simulink model "trucksim_specific_control_with_rule_model"  (R2023b)
settings: Solver=FixedStepAuto  StartTime=0.0  StopTime=25  FixedStep=0.001  RelTol=1e-3  EnableMultiTasking=on
values from neighbouring files (symbols this model uses):
  A = 5    [unlinear_vehicle_Parameters.m]
  Bf = 1.725    [unlinear_vehicle_Parameters.m]
  Br = 1.750    (= 1.75)    [unlinear_vehicle_Parameters.m]
  Cd = 0.4    [unlinear_vehicle_Parameters.m]
  Cs_f = 4302    [unlinear_vehicle_Parameters.m]
  Delta_act_sine_amp = delta_act_sine_amp(j)    [Truck_simulate.m]    (also in unlinear_vehicle_Parameters.m)
  Delta_act_sine_fre = delta_act_sine_fre(k)    [Truck_simulate.m]    (also in unlinear_vehicle_Parameters.m)
  f = 0.01    [unlinear_vehicle_Parameters.m]
  g = 9.8    [Truck_simulate.m]    (also in unlinear_vehicle_Parameters.m)
  He = 0.45    [unlinear_vehicle_Parameters.m]
  hg = 0.781    [unlinear_vehicle_Parameters.m]
  Hp = 0.2    [unlinear_vehicle_Parameters.m]
  I_tire = 0.7    [unlinear_vehicle_Parameters.m]
  Ix = 423.3    [unlinear_vehicle_Parameters.m]
  Iy = 1762.5    [unlinear_vehicle_Parameters.m]
  Iz = 1762.5    [unlinear_vehicle_Parameters.m]
  ks_f = 189000    [unlinear_vehicle_Parameters.m]
  kw = 220000    [unlinear_vehicle_Parameters.m]
  L = 3.140    (= 3.14)    [unlinear_vehicle_Parameters.m]
  Lf = 1.330    (= 1.33)    [unlinear_vehicle_Parameters.m]
  Lr = 3.140 - 1.330    (= 1.81)    [unlinear_vehicle_Parameters.m]
  m = m_sprung + m_load + m_unsprung    (= 10505)    [Truck_simulate.m]    (also in unlinear_vehicle_Parameters.m = 1407.3)
  mb = 1128.5 + 000    (= 1128.5)    [unlinear_vehicle_Parameters.m]
  mw = 139.4 / 2    (= 69.7)    [unlinear_vehicle_Parameters.m]
  p = 1.206    [unlinear_vehicle_Parameters.m]
  r = 0.510    (= 0.51)    [Truck_simulate.m]    (also in unlinear_vehicle_Parameters.m = 0.287)
  T_motor_constant = t_motor_const(i)    [Truck_simulate.m]    (also in unlinear_vehicle_Parameters.m)
  vx0 = 5    [Truck_simulate.m]    (also in unlinear_vehicle_Parameters.m)
  vy0 = 0    [Truck_simulate.m]    (also in unlinear_vehicle_Parameters.m)
  w0 = vx0 / r    (= 9.80392156863)    [Truck_simulate.m]    (also in unlinear_vehicle_Parameters.m = 17.4216027875)
  wz0 = 0    [Truck_simulate.m]    (also in unlinear_vehicle_Parameters.m)
libraries: Solver_SF x1
(part 2 of 4)

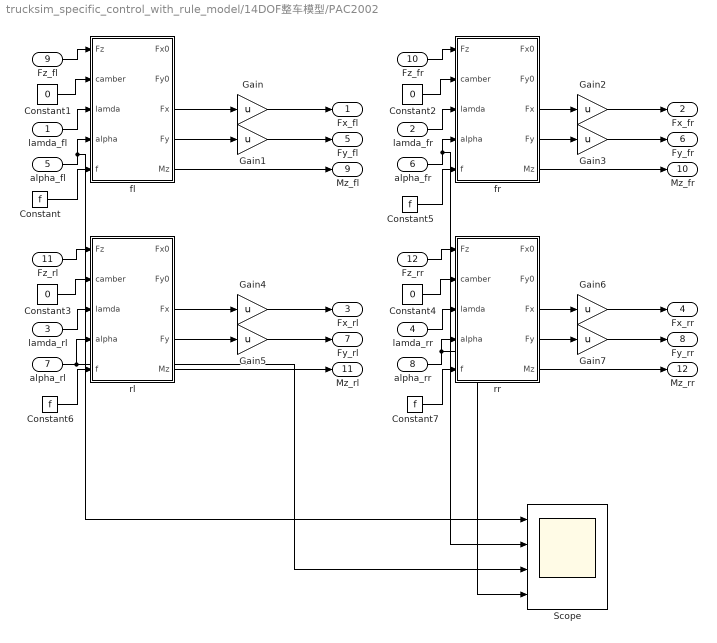
== system trucksim_specific_control_with_rule_model/14DOF整车模型/PAC2002 ==
  lamda_fl : Inport
  lamda_fr : Inport  Port=2
  lamda_rl : Inport  Port=3
  lamda_rr : Inport  Port=4
  alpha_fl : Inport  Port=5
  alpha_fr : Inport  Port=6
  alpha_rl : Inport  Port=7
  alpha_rr : Inport  Port=8
  Fz_fl : Inport  Port=9
  Fz_fr : Inport  Port=10
  Fz_rl : Inport  Port=11
  Fz_rr : Inport  Port=12
  Constant{,5..7} (4 alike) : Constant  Value=f
  Constant{1..4} (4 alike) : Constant  Value=0
  Gain{,1..7} (8 alike) : Gain  Gain=u
  Scope : Scope  NumInputPorts=4
  fl : MATLAB Function  TreatAsAtomicUnit=on
  fr : MATLAB Function  TreatAsAtomicUnit=on
  rl : MATLAB Function  TreatAsAtomicUnit=on
  rr : MATLAB Function  TreatAsAtomicUnit=on
  Fx_fl : Outport
  Fx_fr : Outport  Port=2
  Fx_rl : Outport  Port=3
  Fx_rr : Outport  Port=4
  Fy_fl : Outport  Port=5
  Fy_fr : Outport  Port=6
  Fy_rl : Outport  Port=7
  Fy_rr : Outport  Port=8
  Mz_fl : Outport  Port=9
  Mz_fr : Outport  Port=10
  Mz_rl : Outport  Port=11
  Mz_rr : Outport  Port=12
  wires:
  Constant4/1 -> rr/2(camber)
  Constant3/1 -> rl/2(camber)
  Constant2/1 -> fr/2(camber)
  rr/5(Mz) -> Mz_rr/1
  rl/5(Mz) -> Mz_rl/1
  Fz_rr/1 -> rr/1(Fz)
  alpha_rr/1 -> Scope/4, rr/4(alpha)
  lamda_rr/1 -> rr/3(lamda)
  Fz_rl/1 -> rl/1(Fz)
  alpha_rl/1 -> Scope/3, rl/4(alpha)
  lamda_rl/1 -> rl/3(lamda)
  fr/5(Mz) -> Mz_fr/1
  Fz_fr/1 -> fr/1(Fz)
  alpha_fr/1 -> Scope/2, fr/4(alpha)
  lamda_fr/1 -> fr/3(lamda)
  fl/5(Mz) -> Mz_fl/1
  Constant1/1 -> fl/2(camber)
  Fz_fl/1 -> fl/1(Fz)
  alpha_fl/1 -> Scope/1, fl/4(alpha)
  lamda_fl/1 -> fl/3(lamda)
  fl/3(Fx) -> Gain/1
  fl/4(Fy) -> Gain1/1
  fr/4(Fy) -> Gain3/1
  rr/3(Fx) -> Gain6/1
  rr/4(Fy) -> Gain7/1
  rl/3(Fx) -> Gain4/1
  rl/4(Fy) -> Gain5/1
  fr/3(Fx) -> Gain2/1
  Gain/1 -> Fx_fl/1
  Gain1/1 -> Fy_fl/1
  Gain2/1 -> Fx_fr/1
  Gain3/1 -> Fy_fr/1
  Gain4/1 -> Fx_rl/1
  Gain5/1 -> Fy_rl/1
  Gain6/1 -> Fx_rr/1
  Gain7/1 -> Fy_rr/1
  Constant/1 -> fl/5(f)
  Constant5/1 -> fr/5(f)
  Constant6/1 -> rl/5(f)
  Constant7/1 -> rr/5(f)

== system trucksim_specific_control_with_rule_model/14DOF整车模型/Wheel ==
  T_fl : Inport
  T_fr : Inport  Port=2
  T_rl : Inport  Port=3
  T_rr : Inport  Port=4
  Fx_fl : Inport  Port=5
  Fx_fr : Inport  Port=6
  Fx_rl : Inport  Port=7
  Fx_rr : Inport  Port=8
  Fz_fl : Inport  Port=9
  Fz_fr : Inport  Port=10
  Fz_rl : Inport  Port=11
  Fz_rr : Inport  Port=12
  fl : Subsystem
  fr : Subsystem
  rl : Subsystem
  rr : Subsystem
  w_fl : Outport
  w_fr : Outport  Port=2
  w_rl : Outport  Port=3
  w_rr : Outport  Port=4
  wires:
  rr/1(w_rr) -> w_rr/1
  Fz_rr/1 -> rr/3(Fz_rr)
  Fx_rr/1 -> rr/2(Fx_rr)
  T_rr/1 -> rr/1(T_rr)
  rl/1(w_rl) -> w_rl/1
  Fz_rl/1 -> rl/3(Fz_rl)
  Fx_rl/1 -> rl/2(Fx_rl)
  T_rl/1 -> rl/1(T_rl)
  Fz_fr/1 -> fr/3(Fz_fr)
  Fx_fr/1 -> fr/2(Fx_fr)
  T_fr/1 -> fr/1(T_fr)
  fr/1(w_fr) -> w_fr/1
  fl/1(w_fl) -> w_fl/1
  Fz_fl/1 -> fl/3(Fz_fl)
  Fx_fl/1 -> fl/2(Fx_fl)
  T_fl/1 -> fl/1(T_fl)

== system trucksim_specific_control_with_rule_model/14DOF整车模型/alpha_lamda ==
  vx : Inport
  vy : Inport  Port=2
  wz : Inport  Port=3
  delta_fl : Inport  Port=4
  delta_fr : Inport  Port=5
  delta_rl : Inport  Port=6
  delta_rr : Inport  Port=7
  w_fl : Inport  Port=8
  w_fr : Inport  Port=9
  w_rl : Inport  Port=10
  w_rr : Inport  Port=11
  alpha : Subsystem
  lamda : Subsystem
  lamda_fl : Outport
  lamda_fr : Outport  Port=2
  lamda_rl : Outport  Port=3
  lamda_rr : Outport  Port=4
  alpha_fl : Outport  Port=5
  alpha_fr : Outport  Port=6
  alpha_rl : Outport  Port=7
  alpha_rr : Outport  Port=8
  wires:
  alpha/1(alpha_fl) -> alpha_fl/1
  alpha/2(alpha_fr) -> alpha_fr/1
  alpha/3(alpha_rl) -> alpha_rl/1
  alpha/4(alpha_rr) -> alpha_rr/1
  vx/1 -> lamda/1(vx), alpha/1(vx)
  vy/1 -> lamda/2(vy), alpha/2(vy)
  wz/1 -> lamda/3(wz), alpha/3(wz)
  delta_fl/1 -> lamda/4(delta_fl), alpha/4(delta_fl)
  delta_fr/1 -> lamda/5(delta_fr), alpha/5(delta_fr)
  w_fl/1 -> lamda/6(w_fl)
  w_fr/1 -> lamda/7(w_fr)
  w_rl/1 -> lamda/8(w_rl)
  w_rr/1 -> lamda/9(w_rr)
  lamda/1(lamda_fl) -> lamda_fl/1
  lamda/2(lamda_fr) -> lamda_fr/1
  lamda/4(lamda_rr) -> lamda_rr/1
  lamda/3(lamda_rl) -> lamda_rl/1
  delta_rl/1 -> lamda/10(delta_rl), alpha/6(delta_rl)
  delta_rr/1 -> lamda/11(delta_rr), alpha/7(delta_rr)

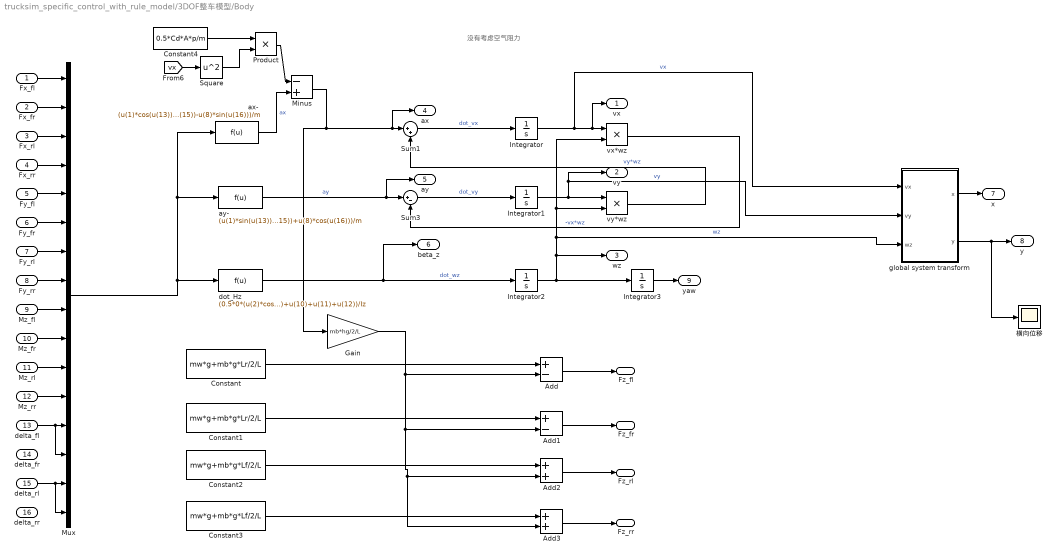
== system trucksim_specific_control_with_rule_model/3DOF整车模型/Body ==
  note: 没有考虑空气阻力
  Fx_fl : Inport
  Fx_fr : Inport  Port=2
  Fx_rl : Inport  Port=3
  Fx_rr : Inport  Port=4
  Fy_fl : Inport  Port=5
  Fy_fr : Inport  Port=6
  Fy_rl : Inport  Port=7
  Fy_rr : Inport  Port=8
  Mz_fl : Inport  Port=9
  Mz_fr : Inport  Port=10
  Mz_rl : Inport  Port=11
  Mz_rr : Inport  Port=12
  delta_fl : Inport  Port=13
  delta_fr : Inport  Port=14
  delta_rl : Inport  Port=15
  delta_rr : Inport  Port=16
  Add : Sum  Inputs=+-
  Add1 : Sum  Inputs=+-
  Add2 : Sum
  Add3 : Sum
  Constant : Constant  Value=mw*g+mb*g*Lr/2/L
  Constant1 : Constant  Value=mw*g+mb*g*Lr/2/L
  Constant2 : Constant  Value=mw*g+mb*g*Lf/2/L
  Constant3 : Constant  Value=mw*g+mb*g*Lf/2/L
  Constant4 : Constant  Value=0.5*Cd*A*p/m
  Gain : Gain  Gain=mb*hg/2/L
  Integrator : Integrator  InitialCondition=vx0  LimitOutput=on  LowerSaturationLimit=0
  Integrator1 : Integrator  InitialCondition=vy0
  Integrator2 : Integrator  InitialCondition=wz0
  Integrator3 : Integrator
  Minus : Sum  Inputs=-+
  Mux : Mux  Inputs=16
  Product : Product
  Square : Math  Operator=square
  Sum1 : Sum  Inputs=|++
  Sum3 : Sum  Inputs=|+-
  ax- : Fcn  Expr=(u(1)*cos(u(13))+u(2)*cos(u(14))-u(5)*sin(u(13))-u(6)*sin(u(14))+u(3)*cos(u(15))+u(4)*cos(u(16))-u(7)*sin(u(15))-u(8)*sin(u(16)))/m
  ay- : Fcn  Expr=(u(1)*sin(u(13))+u(2)*sin(u(14))+u(5)*cos(u(13))+u(6)*cos(u(14))+u(3)*sin(u(15))+u(4)*sin(u(16))+u(7)*cos(u(15))+u(8)*cos(u(16)))/m
  dot_Hz : Fcn  Expr=(0.5*0*(u(2)*cos(u(14))-u(1)*cos(u(13))-u(6)*sin(u(14))+u(5)*sin(u(13)))+0.5*0*(u(4)*cos(u(16))-u(3)*cos(u(15))-u(8)*sin(u(16))+u(7)*sin(u(15)))+Lf*(u(1)*sin(u(13))+u(5)*cos(u(13))+u(2)*sin(u(14))+u(6)*cos(u(14)))-Lr*(u(3)*sin(u(15))+u(7)*cos(u(15))+u(4)*sin(u(16))+u(8)*cos(u(16)))+u(9)+u(10)+u(11)+u(12))/Iz
  global system transform : Subsystem
  vx*wz : Product
  vy*wz : Product
  横向位移 : Scope
  vx : Outport
  vy : Outport  Port=2
  wz : Outport  Port=3
  ax : Outport  Port=4
  ay : Outport  Port=5
  beta_z : Outport  Port=6
  x : Outport  Port=7
  y : Outport  Port=8
  yaw : Outport  Port=9
  Fz_fl : Outport  Port=10
  Fz_fr : Outport  Port=11
  Fz_rl : Outport  Port=12
  Fz_rr : Outport  Port=13
  wires:
  global system transform/2(y) -> y/1, 横向位移/1
  global system transform/1(x) -> x/1
  Mux/1 -> dot_Hz/1, ay-/1, ax-/1
  delta_fl/1 -> Mux/14, Mux/13
  Mz_rr/1 -> Mux/12
  Mz_rl/1 -> Mux/11
  Mz_fr/1 -> Mux/10
  Mz_fl/1 -> Mux/9
  Fy_rr/1 -> Mux/8
  Fy_rl/1 -> Mux/7
  Fy_fr/1 -> Mux/6
  Fy_fl/1 -> Mux/5
  Fx_rr/1 -> Mux/4
  Fx_rl/1 -> Mux/3
  Fx_fr/1 -> Mux/2
  Fx_fl/1 -> Mux/1
  Sum1/1 -> Integrator/1  "dot_vx"
  Integrator/1 -> vx/1, vx*wz/1, global system transform/1(vx)  "vx"
  Integrator1/1 -> global system transform/2(vy), vy/1, vy*wz/1  "vy"
  Sum3/1 -> Integrator1/1  "dot_vy"
  dot_Hz/1 -> beta_z/1, Integrator2/1  "dot_wz"
  Integrator2/1 -> Integrator3/1, global system transform/3(wz), vy*wz/2, vx*wz/2, wz/1  "wz"
  ay-/1 -> ay/1, Sum3/1  "ay"
  vy*wz/1 -> Sum1/2  "vy*wz"
  vx*wz/1 -> Sum3/2  "-vx*wz"
  Constant/1 -> Add/1
  Gain/1 -> Add3/2, Add2/2, Add1/2, Add/2
  Add/1 -> Fz_fl/1
  Constant1/1 -> Add1/1
  Add1/1 -> Fz_fr/1
  Constant2/1 -> Add2/1
  Add2/1 -> Fz_rl/1
  Constant3/1 -> Add3/1
  Add3/1 -> Fz_rr/1
  Constant4/1 -> Product/1
  Square/1 -> Product/2
  [vx] -> Square/1
  Product/1 -> Minus/1
  ax-/1 -> Minus/2  "ax"
  Minus/1 -> Gain/1, ax/1, Sum1/1
  delta_rl/1 -> Mux/16, Mux/15
  Integrator3/1 -> yaw/1

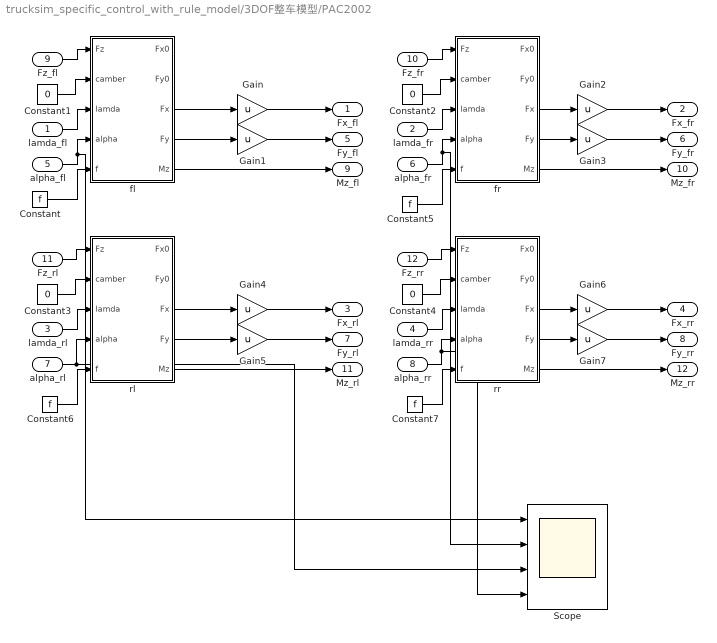
== system trucksim_specific_control_with_rule_model/3DOF整车模型/PAC2002 ==
  lamda_fl : Inport
  lamda_fr : Inport  Port=2
  lamda_rl : Inport  Port=3
  lamda_rr : Inport  Port=4
  alpha_fl : Inport  Port=5
  alpha_fr : Inport  Port=6
  alpha_rl : Inport  Port=7
  alpha_rr : Inport  Port=8
  Fz_fl : Inport  Port=9
  Fz_fr : Inport  Port=10
  Fz_rl : Inport  Port=11
  Fz_rr : Inport  Port=12
  Constant{,5..7} (4 alike) : Constant  Value=f
  Constant{1..4} (4 alike) : Constant  Value=0
  Gain{,1..7} (8 alike) : Gain  Gain=u
  Scope : Scope  NumInputPorts=4
  fl : MATLAB Function  TreatAsAtomicUnit=on
  fr : MATLAB Function  TreatAsAtomicUnit=on
  rl : MATLAB Function  TreatAsAtomicUnit=on
  rr : MATLAB Function  TreatAsAtomicUnit=on
  Fx_fl : Outport
  Fx_fr : Outport  Port=2
  Fx_rl : Outport  Port=3
  Fx_rr : Outport  Port=4
  Fy_fl : Outport  Port=5
  Fy_fr : Outport  Port=6
  Fy_rl : Outport  Port=7
  Fy_rr : Outport  Port=8
  Mz_fl : Outport  Port=9
  Mz_fr : Outport  Port=10
  Mz_rl : Outport  Port=11
  Mz_rr : Outport  Port=12
  wires:
  Constant4/1 -> rr/2(camber)
  Constant3/1 -> rl/2(camber)
  Constant2/1 -> fr/2(camber)
  rr/5(Mz) -> Mz_rr/1
  rl/5(Mz) -> Mz_rl/1
  Fz_rr/1 -> rr/1(Fz)
  alpha_rr/1 -> Scope/4, rr/4(alpha)
  lamda_rr/1 -> rr/3(lamda)
  Fz_rl/1 -> rl/1(Fz)
  alpha_rl/1 -> Scope/3, rl/4(alpha)
  lamda_rl/1 -> rl/3(lamda)
  fr/5(Mz) -> Mz_fr/1
  Fz_fr/1 -> fr/1(Fz)
  alpha_fr/1 -> Scope/2, fr/4(alpha)
  lamda_fr/1 -> fr/3(lamda)
  fl/5(Mz) -> Mz_fl/1
  Constant1/1 -> fl/2(camber)
  Fz_fl/1 -> fl/1(Fz)
  alpha_fl/1 -> Scope/1, fl/4(alpha)
  lamda_fl/1 -> fl/3(lamda)
  fl/3(Fx) -> Gain/1
  fl/4(Fy) -> Gain1/1
  fr/4(Fy) -> Gain3/1
  rr/3(Fx) -> Gain6/1
  rr/4(Fy) -> Gain7/1
  rl/3(Fx) -> Gain4/1
  rl/4(Fy) -> Gain5/1
  fr/3(Fx) -> Gain2/1
  Gain/1 -> Fx_fl/1
  Gain1/1 -> Fy_fl/1
  Gain2/1 -> Fx_fr/1
  Gain3/1 -> Fy_fr/1
  Gain4/1 -> Fx_rl/1
  Gain5/1 -> Fy_rl/1
  Gain6/1 -> Fx_rr/1
  Gain7/1 -> Fy_rr/1
  Constant/1 -> fl/5(f)
  Constant5/1 -> fr/5(f)
  Constant6/1 -> rl/5(f)
  Constant7/1 -> rr/5(f)

== system trucksim_specific_control_with_rule_model/3DOF整车模型/Wheel ==
  T_fl : Inport
  T_fr : Inport  Port=2
  T_rl : Inport  Port=3
  T_rr : Inport  Port=4
  Fx_fl : Inport  Port=5
  Fx_fr : Inport  Port=6
  Fx_rl : Inport  Port=7
  Fx_rr : Inport  Port=8
  Fz_fl : Inport  Port=9
  Fz_fr : Inport  Port=10
  Fz_rl : Inport  Port=11
  Fz_rr : Inport  Port=12
  fl : Subsystem
  fr : Subsystem
  rl : Subsystem
  rr : Subsystem
  w_fl : Outport
  w_fr : Outport  Port=2
  w_rl : Outport  Port=3
  w_rr : Outport  Port=4
  wires:
  T_fl/1 -> fl/1(T_fl)
  Fx_fl/1 -> fl/2(Fx_fl)
  Fz_fl/1 -> fl/3(Fz_fl)
  fl/1(w_fl) -> w_fl/1
  fr/1(w_fr) -> w_fr/1
  T_fr/1 -> fr/1(T_fr)
  Fx_fr/1 -> fr/2(Fx_fr)
  Fz_fr/1 -> fr/3(Fz_fr)
  T_rl/1 -> rl/1(T_rl)
  Fx_rl/1 -> rl/2(Fx_rl)
  Fz_rl/1 -> rl/3(Fz_rl)
  rl/1(w_rl) -> w_rl/1
  T_rr/1 -> rr/1(T_rr)
  Fx_rr/1 -> rr/2(Fx_rr)
  Fz_rr/1 -> rr/3(Fz_rr)
  rr/1(w_rr) -> w_rr/1

== system trucksim_specific_control_with_rule_model/3DOF整车模型/alpha_lamda1 ==
  vx : Inport
  vy : Inport  Port=2
  wz : Inport  Port=3
  delta_fl : Inport  Port=4
  delta_fr : Inport  Port=5
  delta_rl : Inport  Port=6
  delta_rr : Inport  Port=7
  w_fl : Inport  Port=8
  w_fr : Inport  Port=9
  w_rl : Inport  Port=10
  w_rr : Inport  Port=11
  alpha : Subsystem
  lamda : Subsystem
  lamda_fl : Outport
  lamda_fr : Outport  Port=2
  lamda_rl : Outport  Port=3
  lamda_rr : Outport  Port=4
  alpha_fl : Outport  Port=5
  alpha_fr : Outport  Port=6
  alpha_rl : Outport  Port=7
  alpha_rr : Outport  Port=8
  wires:
  alpha/1(alpha_fl) -> alpha_fl/1
  alpha/2(alpha_fr) -> alpha_fr/1
  alpha/3(alpha_rl) -> alpha_rl/1
  alpha/4(alpha_rr) -> alpha_rr/1
  vx/1 -> lamda/1(vx), alpha/1(vx)
  vy/1 -> lamda/2(vy), alpha/2(vy)
  wz/1 -> lamda/3(wz), alpha/3(wz)
  delta_fl/1 -> lamda/4(delta_fl), alpha/4(delta_fl)
  delta_fr/1 -> lamda/5(delta_fr), alpha/5(delta_fr)
  w_fl/1 -> lamda/6(w_fl)
  w_fr/1 -> lamda/7(w_fr)
  w_rl/1 -> lamda/8(w_rl)
  w_rr/1 -> lamda/9(w_rr)
  lamda/1(lamda_fl) -> lamda_fl/1
  lamda/2(lamda_fr) -> lamda_fr/1
  lamda/4(lamda_rr) -> lamda_rr/1
  lamda/3(lamda_rl) -> lamda_rl/1
  delta_rl/1 -> lamda/10(delta_rl), alpha/6(delta_rl)
  delta_rr/1 -> lamda/11(delta_rr), alpha/7(delta_rr)

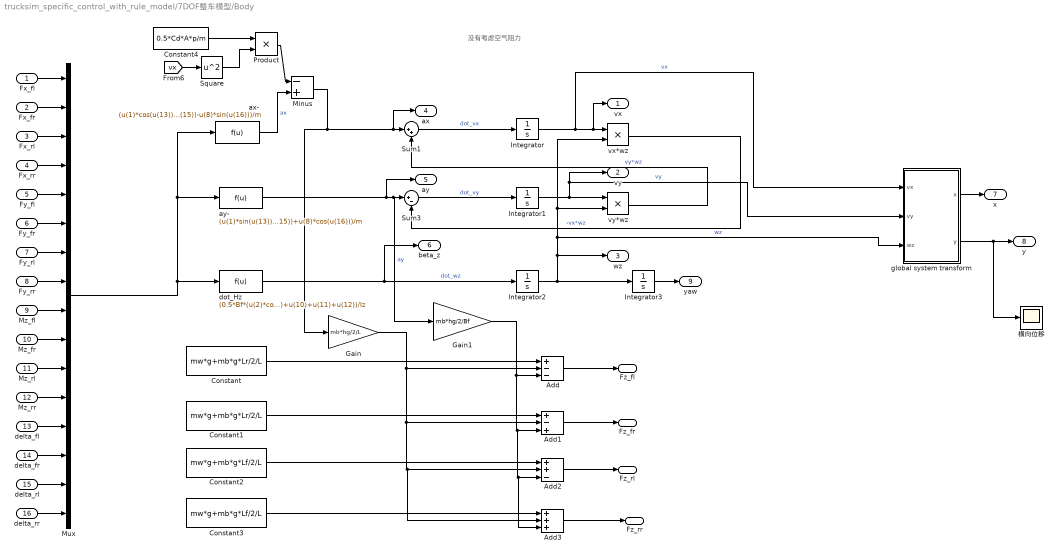
== system trucksim_specific_control_with_rule_model/7DOF整车模型/Body ==
  note: 没有考虑空气阻力
  Fx_fl : Inport
  Fx_fr : Inport  Port=2
  Fx_rl : Inport  Port=3
  Fx_rr : Inport  Port=4
  Fy_fl : Inport  Port=5
  Fy_fr : Inport  Port=6
  Fy_rl : Inport  Port=7
  Fy_rr : Inport  Port=8
  Mz_fl : Inport  Port=9
  Mz_fr : Inport  Port=10
  Mz_rl : Inport  Port=11
  Mz_rr : Inport  Port=12
  delta_fl : Inport  Port=13
  delta_fr : Inport  Port=14
  delta_rl : Inport  Port=15
  delta_rr : Inport  Port=16
  Add : Sum  Inputs=+--
  Add1 : Sum  Inputs=+-+
  Add2 : Sum  Inputs=++-
  Add3 : Sum  Inputs=+++
  Constant : Constant  Value=mw*g+mb*g*Lr/2/L
  Constant1 : Constant  Value=mw*g+mb*g*Lr/2/L
  Constant2 : Constant  Value=mw*g+mb*g*Lf/2/L
  Constant3 : Constant  Value=mw*g+mb*g*Lf/2/L
  Constant4 : Constant  Value=0.5*Cd*A*p/m
  Gain : Gain  Gain=mb*hg/2/L
  Gain1 : Gain  Gain=mb*hg/2/Bf
  Integrator : Integrator  InitialCondition=vx0  LimitOutput=on  LowerSaturationLimit=0
  Integrator1 : Integrator  InitialCondition=vy0
  Integrator2 : Integrator  InitialCondition=wz0
  Integrator3 : Integrator
  Minus : Sum  Inputs=-+
  Mux : Mux  Inputs=16
  Product : Product
  Square : Math  Operator=square
  Sum1 : Sum  Inputs=|++
  Sum3 : Sum  Inputs=|+-
  ax- : Fcn  Expr=(u(1)*cos(u(13))+u(2)*cos(u(14))-u(5)*sin(u(13))-u(6)*sin(u(14))+u(3)*cos(u(15))+u(4)*cos(u(16))-u(7)*sin(u(15))-u(8)*sin(u(16)))/m
  ay- : Fcn  Expr=(u(1)*sin(u(13))+u(2)*sin(u(14))+u(5)*cos(u(13))+u(6)*cos(u(14))+u(3)*sin(u(15))+u(4)*sin(u(16))+u(7)*cos(u(15))+u(8)*cos(u(16)))/m
  dot_Hz : Fcn  Expr=(0.5*Bf*(u(2)*cos(u(14))-u(1)*cos(u(13))-u(6)*sin(u(14))+u(5)*sin(u(13)))+0.5*Br*(u(4)*cos(u(16))-u(3)*cos(u(15))-u(8)*sin(u(16))+u(7)*sin(u(15)))+Lf*(u(1)*sin(u(13))+u(5)*cos(u(13))+u(2)*sin(u(14))+u(6)*cos(u(14)))-Lr*(u(3)*sin(u(15))+u(7)*cos(u(15))+u(4)*sin(u(16))+u(8)*cos(u(16)))+u(9)+u(10)+u(11)+u(12))/Iz
  global system transform : Subsystem
  vx*wz : Product
  vy*wz : Product
  横向位移 : Scope
  vx : Outport
  vy : Outport  Port=2
  wz : Outport  Port=3
  ax : Outport  Port=4
  ay : Outport  Port=5
  beta_z : Outport  Port=6
  x : Outport  Port=7
  y : Outport  Port=8
  yaw : Outport  Port=9
  Fz_fl : Outport  Port=10
  Fz_fr : Outport  Port=11
  Fz_rl : Outport  Port=12
  Fz_rr : Outport  Port=13
  wires:
  global system transform/2(y) -> y/1, 横向位移/1
  global system transform/1(x) -> x/1
  Mux/1 -> dot_Hz/1, ay-/1, ax-/1
  delta_fr/1 -> Mux/14
  delta_fl/1 -> Mux/13
  Mz_rr/1 -> Mux/12
  Mz_rl/1 -> Mux/11
  Mz_fr/1 -> Mux/10
  Mz_fl/1 -> Mux/9
  Fy_rr/1 -> Mux/8
  Fy_rl/1 -> Mux/7
  Fy_fr/1 -> Mux/6
  Fy_fl/1 -> Mux/5
  Fx_rr/1 -> Mux/4
  Fx_rl/1 -> Mux/3
  Fx_fr/1 -> Mux/2
  Fx_fl/1 -> Mux/1
  Sum1/1 -> Integrator/1  "dot_vx"
  Integrator/1 -> vx/1, vx*wz/1, global system transform/1(vx)  "vx"
  Integrator1/1 -> global system transform/2(vy), vy/1, vy*wz/1  "vy"
  Sum3/1 -> Integrator1/1  "dot_vy"
  dot_Hz/1 -> beta_z/1, Integrator2/1  "dot_wz"
  Integrator2/1 -> Integrator3/1, global system transform/3(wz), vy*wz/2, vx*wz/2, wz/1  "wz"
  ay-/1 -> Gain1/1, Sum3/1, ay/1  "ay"
  vy*wz/1 -> Sum1/2  "vy*wz"
  vx*wz/1 -> Sum3/2  "-vx*wz"
  Constant/1 -> Add/1
  Gain/1 -> Add3/2, Add2/2, Add1/2, Add/2
  Gain1/1 -> Add3/3, Add2/3, Add1/3, Add/3
  Add/1 -> Fz_fl/1
  Constant1/1 -> Add1/1
  Add1/1 -> Fz_fr/1
  Constant2/1 -> Add2/1
  Add2/1 -> Fz_rl/1
  Constant3/1 -> Add3/1
  Add3/1 -> Fz_rr/1
  Constant4/1 -> Product/1
  Square/1 -> Product/2
  [vx] -> Square/1
  Product/1 -> Minus/1
  ax-/1 -> Minus/2  "ax"
  Minus/1 -> Gain/1, ax/1, Sum1/1
  delta_rr/1 -> Mux/16
  delta_rl/1 -> Mux/15
  Integrator3/1 -> yaw/1

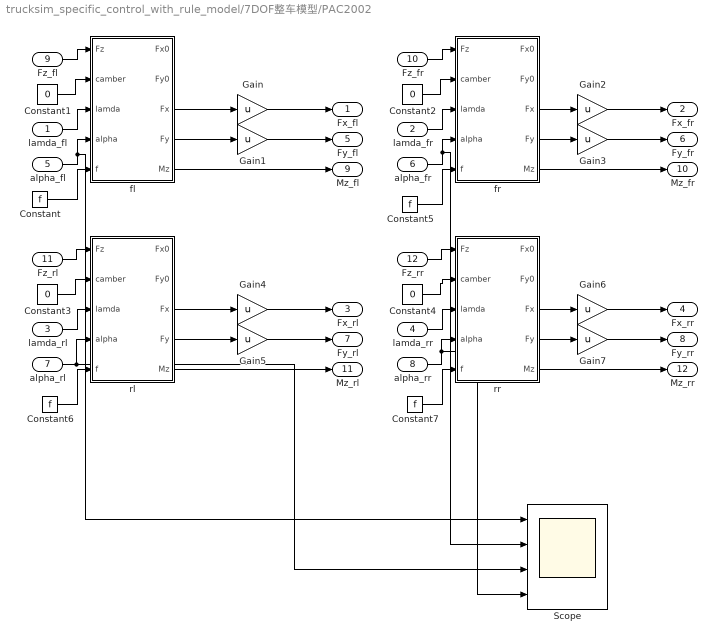
== system trucksim_specific_control_with_rule_model/7DOF整车模型/PAC2002 ==
  lamda_fl : Inport
  lamda_fr : Inport  Port=2
  lamda_rl : Inport  Port=3
  lamda_rr : Inport  Port=4
  alpha_fl : Inport  Port=5
  alpha_fr : Inport  Port=6
  alpha_rl : Inport  Port=7
  alpha_rr : Inport  Port=8
  Fz_fl : Inport  Port=9
  Fz_fr : Inport  Port=10
  Fz_rl : Inport  Port=11
  Fz_rr : Inport  Port=12
  Constant{,5..7} (4 alike) : Constant  Value=f
  Constant{1..4} (4 alike) : Constant  Value=0
  Gain{,1..7} (8 alike) : Gain  Gain=u
  Scope : Scope  NumInputPorts=4
  fl : MATLAB Function  TreatAsAtomicUnit=on
  fr : MATLAB Function  TreatAsAtomicUnit=on
  rl : MATLAB Function  TreatAsAtomicUnit=on
  rr : MATLAB Function  TreatAsAtomicUnit=on
  Fx_fl : Outport
  Fx_fr : Outport  Port=2
  Fx_rl : Outport  Port=3
  Fx_rr : Outport  Port=4
  Fy_fl : Outport  Port=5
  Fy_fr : Outport  Port=6
  Fy_rl : Outport  Port=7
  Fy_rr : Outport  Port=8
  Mz_fl : Outport  Port=9
  Mz_fr : Outport  Port=10
  Mz_rl : Outport  Port=11
  Mz_rr : Outport  Port=12
  wires:
  Constant4/1 -> rr/2(camber)
  Constant3/1 -> rl/2(camber)
  Constant2/1 -> fr/2(camber)
  rr/5(Mz) -> Mz_rr/1
  rl/5(Mz) -> Mz_rl/1
  Fz_rr/1 -> rr/1(Fz)
  alpha_rr/1 -> rr/4(alpha), Scope/4
  lamda_rr/1 -> rr/3(lamda)
  Fz_rl/1 -> rl/1(Fz)
  alpha_rl/1 -> Scope/3, rl/4(alpha)
  lamda_rl/1 -> rl/3(lamda)
  fr/5(Mz) -> Mz_fr/1
  Fz_fr/1 -> fr/1(Fz)
  alpha_fr/1 -> Scope/2, fr/4(alpha)
  lamda_fr/1 -> fr/3(lamda)
  fl/5(Mz) -> Mz_fl/1
  Constant1/1 -> fl/2(camber)
  Fz_fl/1 -> fl/1(Fz)
  alpha_fl/1 -> Scope/1, fl/4(alpha)
  lamda_fl/1 -> fl/3(lamda)
  fl/3(Fx) -> Gain/1
  fl/4(Fy) -> Gain1/1
  fr/4(Fy) -> Gain3/1
  rr/3(Fx) -> Gain6/1
  rr/4(Fy) -> Gain7/1
  rl/3(Fx) -> Gain4/1
  rl/4(Fy) -> Gain5/1
  fr/3(Fx) -> Gain2/1
  Gain/1 -> Fx_fl/1
  Gain1/1 -> Fy_fl/1
  Gain2/1 -> Fx_fr/1
  Gain3/1 -> Fy_fr/1
  Gain4/1 -> Fx_rl/1
  Gain5/1 -> Fy_rl/1
  Gain6/1 -> Fx_rr/1
  Gain7/1 -> Fy_rr/1
  Constant/1 -> fl/5(f)
  Constant5/1 -> fr/5(f)
  Constant6/1 -> rl/5(f)
  Constant7/1 -> rr/5(f)

== system trucksim_specific_control_with_rule_model/7DOF整车模型/Wheel ==
  T_fl : Inport
  T_fr : Inport  Port=2
  T_rl : Inport  Port=3
  T_rr : Inport  Port=4
  Fx_fl : Inport  Port=5
  Fx_fr : Inport  Port=6
  Fx_rl : Inport  Port=7
  Fx_rr : Inport  Port=8
  Fz_fl : Inport  Port=9
  Fz_fr : Inport  Port=10
  Fz_rl : Inport  Port=11
  Fz_rr : Inport  Port=12
  fl : Subsystem
  fr : Subsystem
  rl : Subsystem
  rr : Subsystem
  w_fl : Outport
  w_fr : Outport  Port=2
  w_rl : Outport  Port=3
  w_rr : Outport  Port=4
  wires:
  T_fl/1 -> fl/1(T_fl)
  Fx_fl/1 -> fl/2(Fx_fl)
  Fz_fl/1 -> fl/3(Fz_fl)
  fl/1(w_fl) -> w_fl/1
  fr/1(w_fr) -> w_fr/1
  T_fr/1 -> fr/1(T_fr)
  Fx_fr/1 -> fr/2(Fx_fr)
  Fz_fr/1 -> fr/3(Fz_fr)
  T_rl/1 -> rl/1(T_rl)
  Fx_rl/1 -> rl/2(Fx_rl)
  Fz_rl/1 -> rl/3(Fz_rl)
  rl/1(w_rl) -> w_rl/1
  T_rr/1 -> rr/1(T_rr)
  Fx_rr/1 -> rr/2(Fx_rr)
  Fz_rr/1 -> rr/3(Fz_rr)
  rr/1(w_rr) -> w_rr/1

== system trucksim_specific_control_with_rule_model/7DOF整车模型/alpha_lamda1 ==
  vx : Inport
  vy : Inport  Port=2
  wz : Inport  Port=3
  delta_fl : Inport  Port=4
  delta_fr : Inport  Port=5
  delta_rl : Inport  Port=6
  delta_rr : Inport  Port=7
  w_fl : Inport  Port=8
  w_fr : Inport  Port=9
  w_rl : Inport  Port=10
  w_rr : Inport  Port=11
  alpha : Subsystem
  lamda : Subsystem
  lamda_fl : Outport
  lamda_fr : Outport  Port=2
  lamda_rl : Outport  Port=3
  lamda_rr : Outport  Port=4
  alpha_fl : Outport  Port=5
  alpha_fr : Outport  Port=6
  alpha_rl : Outport  Port=7
  alpha_rr : Outport  Port=8
  wires:
  alpha/1(alpha_fl) -> alpha_fl/1
  alpha/2(alpha_fr) -> alpha_fr/1
  alpha/3(alpha_rl) -> alpha_rl/1
  alpha/4(alpha_rr) -> alpha_rr/1
  vx/1 -> lamda/1(vx), alpha/1(vx)
  vy/1 -> lamda/2(vy), alpha/2(vy)
  wz/1 -> lamda/3(wz), alpha/3(wz)
  delta_fl/1 -> lamda/4(delta_fl), alpha/4(delta_fl)
  delta_fr/1 -> lamda/5(delta_fr), alpha/5(delta_fr)
  w_fl/1 -> lamda/6(w_fl)
  w_fr/1 -> lamda/7(w_fr)
  w_rl/1 -> lamda/8(w_rl)
  w_rr/1 -> lamda/9(w_rr)
  lamda/1(lamda_fl) -> lamda_fl/1
  lamda/2(lamda_fr) -> lamda_fr/1
  lamda/4(lamda_rr) -> lamda_rr/1
  lamda/3(lamda_rl) -> lamda_rl/1
  delta_rl/1 -> lamda/10(delta_rl), alpha/6(delta_rl)
  delta_rr/1 -> lamda/11(delta_rr), alpha/7(delta_rr)

== system trucksim_specific_control_with_rule_model/14DOF整车模型/Body/Suspension_Z ==
  ddot_phi : Inport
  ddot_theta : Inport  Port=2
  ddot_zb : Inport  Port=3
  Zroad : Inport  Port=4
  Demux : Demux
  Integrator{,1..3} (4 alike) : Integrator
  fl : Subsystem
  fr : Subsystem
  rl : Subsystem
  rr : Subsystem
  zb_to_zs : Subsystem
  Fzs_fl : Outport
  Fzs_fr : Outport  Port=2
  Fzs_rl : Outport  Port=3
  Fzs_rr : Outport  Port=4
  Fzw_fl : Outport  Port=5
  Fzw_fr : Outport  Port=6
  Fzw_rl : Outport  Port=7
  Fzw_rr : Outport  Port=8
  wires:
  ddot_phi/1 -> zb_to_zs/1(ddot_phi)
  ddot_theta/1 -> zb_to_zs/2(ddot_theta)
  ddot_zb/1 -> zb_to_zs/3(ddot_zb)
  fl/1(Fzs_fl) -> Fzs_fl/1
  zb_to_zs/1(dot_Zs_fl) -> Integrator/1, fl/1(dot_Zs_fl)
  Zroad/1 -> Demux/1
  Integrator/1 -> fl/3(Zs_fl)
  fr/1(Fzs_fr) -> Fzs_fr/1
  zb_to_zs/2(dot_Zs_fr) -> fr/1(dot_Zs_fr), Integrator1/1
  Demux/2 -> fr/2(Z_road_fr)
  Integrator1/1 -> fr/3(Zs_fr)
  fl/2(Fzw_fl) -> Fzw_fl/1
  fr/2(Fzw_fr) -> Fzw_fr/1
  zb_to_zs/3(dot_Zs_rl) -> rl/1(dot_Zs_rl), Integrator2/1
  Integrator2/1 -> rl/3(Zs_rl)
  Demux/3 -> rl/2(Z_road_rl)
  rl/1(Fzs_rl) -> Fzs_rl/1
  rl/2(Fzw_fl) -> Fzw_rl/1
  zb_to_zs/4(dot_Zs_rr) -> Integrator3/1, rr/1(dot_Zs_rr)
  Demux/4 -> rr/2(Z_road_rr)
  Integrator3/1 -> rr/3(Zs_rr)
  rr/1(Fzs_rr) -> Fzs_rr/1
  rr/2(Fzw_fl) -> Fzw_rr/1
  Demux/1 -> fl/2(Z_road_fl)

== system trucksim_specific_control_with_rule_model/14DOF整车模型/Body/global system transform ==
  vx : Inport
  vy : Inport  Port=2
  wz : Inport  Port=3
  Add : Sum  Inputs=|+-
  Add1 : Sum  Inputs=|++
  Integrator10 : Integrator
  Integrator8 : Integrator
  Integrator9 : Integrator
  Trigonometric Function1 : Trigonometry
  Trigonometric Function2 : Trigonometry  Operator=cos
  vx*cosr : Product
  vx*sinr : Product
  vy*cosr : Product
  vy*sinr : Product
  x : Outport
  y : Outport  Port=2
  wires:
  Add/1 -> Integrator10/1
  Trigonometric Function2/1 -> vy*cosr/2, vx*cosr/2
  vy*sinr/1 -> Add/2
  vx/1 -> vx*sinr/1, vx*cosr/1
  wz/1 -> Integrator8/1
  vy/1 -> vy*sinr/1, vy*cosr/1
  Integrator9/1 -> y/1
  Integrator10/1 -> x/1
  Integrator8/1 -> Trigonometric Function2/1, Trigonometric Function1/1  "r"
  Trigonometric Function1/1 -> vx*sinr/2, vy*sinr/2
  vx*cosr/1 -> Add/1
  vx*sinr/1 -> Add1/1
  Add1/1 -> Integrator9/1
  vy*cosr/1 -> Add1/2

== system trucksim_specific_control_with_rule_model/14DOF整车模型/Wheel/fl ==
  T_fl : Inport
  Fx_fl : Inport  Port=2
  Fz_fl : Inport  Port=3
  Add : Sum  Inputs=+--
  Constant : Constant  Value=I_tire
  Divide : Product  Inputs=*/
  Gain : Gain  Gain=r
  Gain1 : Gain  Gain=r*f
  Integrator : Integrator  InitialCondition=w0
  w_fl : Outport
  wires:
  Integrator/1 -> w_fl/1
  Divide/1 -> Integrator/1  "dot_w"
  Constant/1 -> Divide/2
  Add/1 -> Divide/1
  Gain1/1 -> Add/3
  T_fl/1 -> Add/1
  Fz_fl/1 -> Gain1/1
  Fx_fl/1 -> Gain/1
  Gain/1 -> Add/2

== system trucksim_specific_control_with_rule_model/14DOF整车模型/Wheel/fr ==
  T_fr : Inport
  Fx_fr : Inport  Port=2
  Fz_fr : Inport  Port=3
  Add : Sum  Inputs=+--
  Constant : Constant  Value=I_tire
  Divide : Product  Inputs=*/
  Gain : Gain  Gain=r
  Gain1 : Gain  Gain=r*f
  Integrator : Integrator  InitialCondition=w0
  w_fr : Outport
  wires:
  Fx_fr/1 -> Gain/1
  Fz_fr/1 -> Gain1/1
  T_fr/1 -> Add/1
  Gain/1 -> Add/2
  Add/1 -> Divide/1
  Constant/1 -> Divide/2
  Divide/1 -> Integrator/1  "dot_w"
  Integrator/1 -> w_fr/1
  Gain1/1 -> Add/3

== system trucksim_specific_control_with_rule_model/14DOF整车模型/Wheel/rl ==
  T_rl : Inport
  Fx_rl : Inport  Port=2
  Fz_rl : Inport  Port=3
  Add : Sum  Inputs=+--
  Constant : Constant  Value=I_tire
  Divide : Product  Inputs=*/
  Gain : Gain  Gain=r
  Gain1 : Gain  Gain=r*f
  Integrator : Integrator  InitialCondition=w0
  w_rl : Outport
  wires:
  Fx_rl/1 -> Gain/1
  Fz_rl/1 -> Gain1/1
  T_rl/1 -> Add/1
  Gain/1 -> Add/2
  Add/1 -> Divide/1
  Constant/1 -> Divide/2
  Divide/1 -> Integrator/1  "dot_w"
  Integrator/1 -> w_rl/1
  Gain1/1 -> Add/3

== system trucksim_specific_control_with_rule_model/14DOF整车模型/Wheel/rr ==
  T_rr : Inport
  Fx_rr : Inport  Port=2
  Fz_rr : Inport  Port=3
  Add : Sum  Inputs=+--
  Constant : Constant  Value=I_tire
  Divide : Product  Inputs=*/
  Gain : Gain  Gain=r
  Gain1 : Gain  Gain=r*f
  Integrator : Integrator  InitialCondition=w0
  w_rr : Outport
  wires:
  Integrator/1 -> w_rr/1
  Divide/1 -> Integrator/1  "dot_w"
  Constant/1 -> Divide/2
  Add/1 -> Divide/1
  Gain/1 -> Add/2
  T_rr/1 -> Add/1
  Fz_rr/1 -> Gain1/1
  Fx_rr/1 -> Gain/1
  Gain1/1 -> Add/3

== system trucksim_specific_control_with_rule_model/14DOF整车模型/alpha_lamda/alpha ==
  vx : Inport
  vy : Inport  Port=2
  wz : Inport  Port=3
  delta_fl : Inport  Port=4
  delta_fr : Inport  Port=5
  delta_rl : Inport  Port=6
  delta_rr : Inport  Port=7
  Gain{,1..3} (4 alike) : Gain  Gain=-1
  fl : Subsystem
  fr : Subsystem
  rl : Subsystem
  rr : Subsystem
  alpha_fl : Outport
  alpha_fr : Outport  Port=2
  alpha_rl : Outport  Port=3
  alpha_rr : Outport  Port=4
  wires:
  Gain3/1 -> alpha_rr/1
  rr/1(alpha_rr) -> Gain3/1
  Gain2/1 -> alpha_fr/1
  fr/1(alpha_fr) -> Gain2/1
  Gain1/1 -> alpha_rl/1
  rl/1(alpha_rl) -> Gain1/1
  Gain/1 -> alpha_fl/1
  fl/1(alpha_fl) -> Gain/1
  wz/1 -> fl/3(wz), rr/3(wz), fr/3(wz), rl/3(wz)
  vx/1 -> rr/1(vx), fr/1(vx), fl/1(vx), rl/1(vx)
  vy/1 -> rr/2(vy), fr/2(vy), fl/2(vy), rl/2(vy)
  delta_fl/1 -> fl/4(delta_fl)
  delta_fr/1 -> fr/4(delta_fr)
  delta_rl/1 -> rl/4(delta_rl)
  delta_rr/1 -> rr/4(delta_rr)

== system trucksim_specific_control_with_rule_model/14DOF整车模型/alpha_lamda/lamda ==
  vx : Inport
  vy : Inport  Port=2
  wz : Inport  Port=3
  delta_fl : Inport  Port=4
  delta_fr : Inport  Port=5
  w_fl : Inport  Port=6
  w_fr : Inport  Port=7
  w_rl : Inport  Port=8
  w_rr : Inport  Port=9
  delta_rl : Inport  Port=10
  delta_rr : Inport  Port=11
  fl : Subsystem
  fr : Subsystem
  rl : Subsystem
  rr : Subsystem
  lamda_fl : Outport
  lamda_fr : Outport  Port=2
  lamda_rl : Outport  Port=3
  lamda_rr : Outport  Port=4
  wires:
  fl/1(lamda_fl) -> lamda_fl/1
  rl/1(lamda_rl) -> lamda_rl/1
  w_fl/1 -> fl/1(w_fl)
  wz/1 -> rl/2(wz), rr/2(wz), fr/2(wz), fl/2(wz)
  vx/1 -> rl/3(vx), rr/3(vx), fr/3(vx), fl/3(vx)
  vy/1 -> rl/4(vy), rr/4(vy), fr/4(vy), fl/4(vy)
  delta_fl/1 -> fl/5(delta_fl)
  delta_fr/1 -> fr/5(delta_fr)
  w_fr/1 -> fr/1(w_fr)
  w_rr/1 -> rr/1(w_rr)
  w_rl/1 -> rl/1(w_rl)
  rr/1(lamda_rr) -> lamda_rr/1
  fr/1(lamda_fr) -> lamda_fr/1
  delta_rl/1 -> rl/5(delta_rl)
  delta_rr/1 -> rr/5(delta_rr)

== system trucksim_specific_control_with_rule_model/3DOF整车模型/Body/global system transform ==
  vx : Inport
  vy : Inport  Port=2
  wz : Inport  Port=3
  Add : Sum  Inputs=|+-
  Add1 : Sum  Inputs=|++
  Integrator10 : Integrator
  Integrator8 : Integrator
  Integrator9 : Integrator
  Trigonometric Function1 : Trigonometry
  Trigonometric Function2 : Trigonometry  Operator=cos
  vx*cosr : Product
  vx*sinr : Product
  vy*cosr : Product
  vy*sinr : Product
  x : Outport
  y : Outport  Port=2
  wires:
  vy*cosr/1 -> Add1/2
  Add1/1 -> Integrator9/1
  vx*sinr/1 -> Add1/1
  vx*cosr/1 -> Add/1
  Trigonometric Function1/1 -> vy*sinr/2, vx*sinr/2
  Integrator8/1 -> Trigonometric Function1/1, Trigonometric Function2/1  "r"
  Integrator10/1 -> x/1
  Integrator9/1 -> y/1
  vy/1 -> vy*cosr/1, vy*sinr/1
  wz/1 -> Integrator8/1
  vx/1 -> vx*cosr/1, vx*sinr/1
  vy*sinr/1 -> Add/2
  Trigonometric Function2/1 -> vx*cosr/2, vy*cosr/2
  Add/1 -> Integrator10/1

== system trucksim_specific_control_with_rule_model/3DOF整车模型/Wheel/fl ==
  T_fl : Inport
  Fx_fl : Inport  Port=2
  Fz_fl : Inport  Port=3
  Add : Sum  Inputs=+--
  Constant : Constant  Value=I_tire
  Divide : Product  Inputs=*/
  Gain : Gain  Gain=r
  Gain1 : Gain  Gain=r*f
  Integrator : Integrator  InitialCondition=w0
  w_fl : Outport
  wires:
  Gain/1 -> Add/2
  Fx_fl/1 -> Gain/1
  Fz_fl/1 -> Gain1/1
  T_fl/1 -> Add/1
  Gain1/1 -> Add/3
  Add/1 -> Divide/1
  Constant/1 -> Divide/2
  Divide/1 -> Integrator/1  "dot_w"
  Integrator/1 -> w_fl/1

== system trucksim_specific_control_with_rule_model/3DOF整车模型/Wheel/fr ==
  T_fr : Inport
  Fx_fr : Inport  Port=2
  Fz_fr : Inport  Port=3
  Add : Sum  Inputs=+--
  Constant : Constant  Value=I_tire
  Divide : Product  Inputs=*/
  Gain : Gain  Gain=r
  Gain1 : Gain  Gain=r*f
  Integrator : Integrator  InitialCondition=w0
  w_fr : Outport
  wires:
  Gain1/1 -> Add/3
  Integrator/1 -> w_fr/1
  Divide/1 -> Integrator/1  "dot_w"
  Constant/1 -> Divide/2
  Add/1 -> Divide/1
  Gain/1 -> Add/2
  T_fr/1 -> Add/1
  Fz_fr/1 -> Gain1/1
  Fx_fr/1 -> Gain/1

== system trucksim_specific_control_with_rule_model/3DOF整车模型/Wheel/rl ==
  T_rl : Inport
  Fx_rl : Inport  Port=2
  Fz_rl : Inport  Port=3
  Add : Sum  Inputs=+--
  Constant : Constant  Value=I_tire
  Divide : Product  Inputs=*/
  Gain : Gain  Gain=r
  Gain1 : Gain  Gain=r*f
  Integrator : Integrator  InitialCondition=w0
  w_rl : Outport
  wires:
  Gain1/1 -> Add/3
  Integrator/1 -> w_rl/1
  Divide/1 -> Integrator/1  "dot_w"
  Constant/1 -> Divide/2
  Add/1 -> Divide/1
  Gain/1 -> Add/2
  T_rl/1 -> Add/1
  Fz_rl/1 -> Gain1/1
  Fx_rl/1 -> Gain/1

== system trucksim_specific_control_with_rule_model/3DOF整车模型/Wheel/rr ==
  T_rr : Inport
  Fx_rr : Inport  Port=2
  Fz_rr : Inport  Port=3
  Add : Sum  Inputs=+--
  Constant : Constant  Value=I_tire
  Divide : Product  Inputs=*/
  Gain : Gain  Gain=r
  Gain1 : Gain  Gain=r*f
  Integrator : Integrator  InitialCondition=w0
  w_rr : Outport
  wires:
  Gain1/1 -> Add/3
  Fx_rr/1 -> Gain/1
  Fz_rr/1 -> Gain1/1
  T_rr/1 -> Add/1
  Gain/1 -> Add/2
  Add/1 -> Divide/1
  Constant/1 -> Divide/2
  Divide/1 -> Integrator/1  "dot_w"
  Integrator/1 -> w_rr/1

== system trucksim_specific_control_with_rule_model/3DOF整车模型/alpha_lamda1/alpha ==
  vx : Inport
  vy : Inport  Port=2
  wz : Inport  Port=3
  delta_fl : Inport  Port=4
  delta_fr : Inport  Port=5
  delta_rl : Inport  Port=6
  delta_rr : Inport  Port=7
  Gain{,1..3} (4 alike) : Gain  Gain=-1
  fl : Subsystem
  fr : Subsystem
  rl : Subsystem
  rr : Subsystem
  alpha_fl : Outport
  alpha_fr : Outport  Port=2
  alpha_rl : Outport  Port=3
  alpha_rr : Outport  Port=4
  wires:
  Gain3/1 -> alpha_rr/1
  rr/1(alpha_rr) -> Gain3/1
  Gain2/1 -> alpha_fr/1
  fr/1(alpha_fr) -> Gain2/1
  Gain1/1 -> alpha_rl/1
  rl/1(alpha_rl) -> Gain1/1
  Gain/1 -> alpha_fl/1
  fl/1(alpha_fl) -> Gain/1
  wz/1 -> fl/3(wz), rr/3(wz), fr/3(wz), rl/3(wz)
  vx/1 -> rr/1(vx), fr/1(vx), fl/1(vx), rl/1(vx)
  vy/1 -> rr/2(vy), fr/2(vy), fl/2(vy), rl/2(vy)
  delta_fl/1 -> fl/4(delta_fl)
  delta_fr/1 -> fr/4(delta_fr)
  delta_rl/1 -> rl/4(delta_rl)
  delta_rr/1 -> rr/4(delta_rr)

== system trucksim_specific_control_with_rule_model/3DOF整车模型/alpha_lamda1/lamda ==
  vx : Inport
  vy : Inport  Port=2
  wz : Inport  Port=3
  delta_fl : Inport  Port=4
  delta_fr : Inport  Port=5
  w_fl : Inport  Port=6
  w_fr : Inport  Port=7
  w_rl : Inport  Port=8
  w_rr : Inport  Port=9
  delta_rl : Inport  Port=10
  delta_rr : Inport  Port=11
  fl : Subsystem
  fr : Subsystem
  rl : Subsystem
  rr : Subsystem
  lamda_fl : Outport
  lamda_fr : Outport  Port=2
  lamda_rl : Outport  Port=3
  lamda_rr : Outport  Port=4
  wires:
  fl/1(lamda_fl) -> lamda_fl/1
  rl/1(lamda_rl) -> lamda_rl/1
  w_fl/1 -> fl/1(w_fl)
  wz/1 -> rl/2(wz), rr/2(wz), fr/2(wz), fl/2(wz)
  vx/1 -> rl/3(vx), rr/3(vx), fr/3(vx), fl/3(vx)
  vy/1 -> rl/4(vy), rr/4(vy), fr/4(vy), fl/4(vy)
  delta_fl/1 -> fl/5(delta_fl)
  delta_fr/1 -> fr/5(delta_fr)
  w_fr/1 -> fr/1(w_fr)
  w_rr/1 -> rr/1(w_rr)
  w_rl/1 -> rl/1(w_rl)
  rr/1(lamda_rr) -> lamda_rr/1
  fr/1(lamda_fr) -> lamda_fr/1
  delta_rl/1 -> rl/5(delta_rl)
  delta_rr/1 -> rr/5(delta_rr)

== system trucksim_specific_control_with_rule_model/7DOF整车模型/Body/global system transform ==
  vx : Inport
  vy : Inport  Port=2
  wz : Inport  Port=3
  Add : Sum  Inputs=|+-
  Add1 : Sum  Inputs=|++
  Integrator10 : Integrator
  Integrator8 : Integrator
  Integrator9 : Integrator
  Trigonometric Function1 : Trigonometry
  Trigonometric Function2 : Trigonometry  Operator=cos
  vx*cosr : Product
  vx*sinr : Product
  vy*cosr : Product
  vy*sinr : Product
  x : Outport
  y : Outport  Port=2
  wires:
  vy*cosr/1 -> Add1/2
  Add1/1 -> Integrator9/1
  vx*sinr/1 -> Add1/1
  vx*cosr/1 -> Add/1
  Trigonometric Function1/1 -> vy*sinr/2, vx*sinr/2
  Integrator8/1 -> Trigonometric Function1/1, Trigonometric Function2/1  "r"
  Integrator10/1 -> x/1
  Integrator9/1 -> y/1
  vy/1 -> vy*cosr/1, vy*sinr/1
  wz/1 -> Integrator8/1
  vx/1 -> vx*cosr/1, vx*sinr/1
  vy*sinr/1 -> Add/2
  Trigonometric Function2/1 -> vx*cosr/2, vy*cosr/2
  Add/1 -> Integrator10/1

== system trucksim_specific_control_with_rule_model/7DOF整车模型/Wheel/fl ==
  T_fl : Inport
  Fx_fl : Inport  Port=2
  Fz_fl : Inport  Port=3
  Add : Sum  Inputs=+--
  Constant : Constant  Value=I_tire
  Divide : Product  Inputs=*/
  Gain : Gain  Gain=r
  Gain1 : Gain  Gain=r*f
  Integrator : Integrator  InitialCondition=w0
  w_fl : Outport
  wires:
  Gain/1 -> Add/2
  Fx_fl/1 -> Gain/1
  Fz_fl/1 -> Gain1/1
  T_fl/1 -> Add/1
  Gain1/1 -> Add/3
  Add/1 -> Divide/1
  Constant/1 -> Divide/2
  Divide/1 -> Integrator/1  "dot_w"
  Integrator/1 -> w_fl/1

== system trucksim_specific_control_with_rule_model/7DOF整车模型/Wheel/fr ==
  T_fr : Inport
  Fx_fr : Inport  Port=2
  Fz_fr : Inport  Port=3
  Add : Sum  Inputs=+--
  Constant : Constant  Value=I_tire
  Divide : Product  Inputs=*/
  Gain : Gain  Gain=r
  Gain1 : Gain  Gain=r*f
  Integrator : Integrator  InitialCondition=w0
  w_fr : Outport
  wires:
  Gain1/1 -> Add/3
  Integrator/1 -> w_fr/1
  Divide/1 -> Integrator/1  "dot_w"
  Constant/1 -> Divide/2
  Add/1 -> Divide/1
  Gain/1 -> Add/2
  T_fr/1 -> Add/1
  Fz_fr/1 -> Gain1/1
  Fx_fr/1 -> Gain/1

== system trucksim_specific_control_with_rule_model/7DOF整车模型/Wheel/rl ==
  T_rl : Inport
  Fx_rl : Inport  Port=2
  Fz_rl : Inport  Port=3
  Add : Sum  Inputs=+--
  Constant : Constant  Value=I_tire
  Divide : Product  Inputs=*/
  Gain : Gain  Gain=r
  Gain1 : Gain  Gain=r*f
  Integrator : Integrator  InitialCondition=w0
  w_rl : Outport
  wires:
  Gain1/1 -> Add/3
  Integrator/1 -> w_rl/1
  Divide/1 -> Integrator/1  "dot_w"
  Constant/1 -> Divide/2
  Add/1 -> Divide/1
  Gain/1 -> Add/2
  T_rl/1 -> Add/1
  Fz_rl/1 -> Gain1/1
  Fx_rl/1 -> Gain/1

== system trucksim_specific_control_with_rule_model/7DOF整车模型/Wheel/rr ==
  T_rr : Inport
  Fx_rr : Inport  Port=2
  Fz_rr : Inport  Port=3
  Add : Sum  Inputs=+--
  Constant : Constant  Value=I_tire
  Divide : Product  Inputs=*/
  Gain : Gain  Gain=r
  Gain1 : Gain  Gain=r*f
  Integrator : Integrator  InitialCondition=w0
  w_rr : Outport
  wires:
  Gain1/1 -> Add/3
  Fx_rr/1 -> Gain/1
  Fz_rr/1 -> Gain1/1
  T_rr/1 -> Add/1
  Gain/1 -> Add/2
  Add/1 -> Divide/1
  Constant/1 -> Divide/2
  Divide/1 -> Integrator/1  "dot_w"
  Integrator/1 -> w_rr/1

== system trucksim_specific_control_with_rule_model/7DOF整车模型/alpha_lamda1/alpha ==
  vx : Inport
  vy : Inport  Port=2
  wz : Inport  Port=3
  delta_fl : Inport  Port=4
  delta_fr : Inport  Port=5
  delta_rl : Inport  Port=6
  delta_rr : Inport  Port=7
  Gain{,1..3} (4 alike) : Gain  Gain=-1
  fl : Subsystem
  fr : Subsystem
  rl : Subsystem
  rr : Subsystem
  alpha_fl : Outport
  alpha_fr : Outport  Port=2
  alpha_rl : Outport  Port=3
  alpha_rr : Outport  Port=4
  wires:
  Gain3/1 -> alpha_rr/1
  rr/1(alpha_rr) -> Gain3/1
  Gain2/1 -> alpha_fr/1
  fr/1(alpha_fr) -> Gain2/1
  Gain1/1 -> alpha_rl/1
  rl/1(alpha_rl) -> Gain1/1
  Gain/1 -> alpha_fl/1
  fl/1(alpha_fl) -> Gain/1
  wz/1 -> fl/3(wz), rr/3(wz), fr/3(wz), rl/3(wz)
  vx/1 -> rr/1(vx), fr/1(vx), fl/1(vx), rl/1(vx)
  vy/1 -> rr/2(vy), fr/2(vy), fl/2(vy), rl/2(vy)
  delta_fl/1 -> fl/4(delta_fl)
  delta_fr/1 -> fr/4(delta_fr)
  delta_rl/1 -> rl/4(delta_rl)
  delta_rr/1 -> rr/4(delta_rr)

== system trucksim_specific_control_with_rule_model/7DOF整车模型/alpha_lamda1/lamda ==
  vx : Inport
  vy : Inport  Port=2
  wz : Inport  Port=3
  delta_fl : Inport  Port=4
  delta_fr : Inport  Port=5
  w_fl : Inport  Port=6
  w_fr : Inport  Port=7
  w_rl : Inport  Port=8
  w_rr : Inport  Port=9
  delta_rl : Inport  Port=10
  delta_rr : Inport  Port=11
  fl : Subsystem
  fr : Subsystem
  rl : Subsystem
  rr : Subsystem
  lamda_fl : Outport
  lamda_fr : Outport  Port=2
  lamda_rl : Outport  Port=3
  lamda_rr : Outport  Port=4
  wires:
  fl/1(lamda_fl) -> lamda_fl/1
  rl/1(lamda_rl) -> lamda_rl/1
  w_fl/1 -> fl/1(w_fl)
  wz/1 -> rl/2(wz), rr/2(wz), fr/2(wz), fl/2(wz)
  vx/1 -> rl/3(vx), rr/3(vx), fr/3(vx), fl/3(vx)
  vy/1 -> rl/4(vy), rr/4(vy), fr/4(vy), fl/4(vy)
  delta_fl/1 -> fl/5(delta_fl)
  delta_fr/1 -> fr/5(delta_fr)
  w_fr/1 -> fr/1(w_fr)
  w_rr/1 -> rr/1(w_rr)
  w_rl/1 -> rl/1(w_rl)
  rr/1(lamda_rr) -> lamda_rr/1
  fr/1(lamda_fr) -> lamda_fr/1
  delta_rl/1 -> rl/5(delta_rl)
  delta_rr/1 -> rr/5(delta_rr)

== system trucksim_specific_control_with_rule_model/14DOF整车模型/Body/Suspension_Z/fl ==
  dot_Zs_fl : Inport
  Z_road_fl : Inport  Port=2
  Zs_fl : Inport  Port=3
  . : Gain  Gain=ks_f
  .1 : Gain  Gain=Cs_f
  Add : Sum  Inputs=-+
  Add{1..2,4,6} (4 alike) : Sum  Inputs=+-
  Add3 : Sum
  Add5 : Sum
  Add7 : Sum
  Constant1 : Constant  Value=0.5*mb*g*Lr/(Lf+Lr)
  Constant2 : Constant  Value=0.5*mb*g*Lr/(Lf+Lr)+mw*g
  Gain : Gain  Gain=1/mw
  Gain1 : Gain  Gain=kw
  Gain2 : Gain  Gain=kw
  Integrator : Integrator
  Integrator1 : Integrator
  Fzs_fl : Outport
  Fzw_fl : Outport  Port=2
  wires:
  Add5/1 -> Fzs_fl/1
  Constant1/1 -> Add5/2
  Integrator/1 -> Add2/1, Integrator1/1
  Integrator1/1 -> Add6/2, Add1/1, Add/1  "Zw_fl"
  Z_road_fl/1 -> Add/2, Add6/1
  Add/1 -> Gain1/1
  Gain1/1 -> Add4/1  "F2zw_fl"
  Zs_fl/1 -> Add1/2
  Add1/1 -> ./1
  dot_Zs_fl/1 -> Add2/2
  Add2/1 -> .1/1
  ./1 -> Add3/1
  .1/1 -> Add3/2
  Add3/1 -> Add4/2, Add5/1  "F2zs_fl"
  Add4/1 -> Gain/1
  Gain/1 -> Integrator/1
  Add6/1 -> Gain2/1
  Gain2/1 -> Add7/1  "F2zw_fl"
  Constant2/1 -> Add7/2
  Add7/1 -> Fzw_fl/1

== system trucksim_specific_control_with_rule_model/14DOF整车模型/Body/Suspension_Z/fr ==
  dot_Zs_fr : Inport
  Z_road_fr : Inport  Port=2
  Zs_fr : Inport  Port=3
  . : Gain  Gain=ks_f
  .1 : Gain  Gain=Cs_f
  Add : Sum  Inputs=-+
  Add{1..2,4,6} (4 alike) : Sum  Inputs=+-
  Add3 : Sum
  Add5 : Sum
  Add7 : Sum
  Constant1 : Constant  Value=0.5*mb*g*Lr/(Lf+Lr)
  Constant2 : Constant  Value=0.5*mb*g*Lr/(Lf+Lr)+mw*g
  Gain : Gain  Gain=1/mw
  Gain1 : Gain  Gain=kw
  Gain2 : Gain  Gain=kw
  Integrator : Integrator
  Integrator1 : Integrator
  Fzs_fr : Outport
  Fzw_fr : Outport  Port=2
  wires:
  Add5/1 -> Fzs_fr/1
  Constant1/1 -> Add5/2
  Add3/1 -> Add4/2, Add5/1  "F2zs_fl"
  Gain/1 -> Integrator/1
  Add4/1 -> Gain/1
  .1/1 -> Add3/2
  ./1 -> Add3/1
  Add2/1 -> .1/1
  dot_Zs_fr/1 -> Add2/2
  Add1/1 -> ./1
  Zs_fr/1 -> Add1/2
  Add/1 -> Gain1/1
  Integrator1/1 -> Add/1, Add1/1, Add6/2  "Zw_fl"
  Integrator/1 -> Integrator1/1, Add2/1
  Z_road_fr/1 -> Add6/1, Add/2
  Gain1/1 -> Add4/1  "F2zw_fl"
  Add6/1 -> Gain2/1
  Gain2/1 -> Add7/1  "F2zw_fl"
  Constant2/1 -> Add7/2
  Add7/1 -> Fzw_fr/1

== system trucksim_specific_control_with_rule_model/14DOF整车模型/Body/Suspension_Z/rl ==
  dot_Zs_rl : Inport
  Z_road_rl : Inport  Port=2
  Zs_rl : Inport  Port=3
  . : Gain  Gain=ks_f
  .1 : Gain  Gain=Cs_f
  Add : Sum  Inputs=-+
  Add{1..2,4,6} (4 alike) : Sum  Inputs=+-
  Add3 : Sum
  Add5 : Sum
  Add7 : Sum
  Constant1 : Constant  Value=0.5*mb*g*Lf/(Lf+Lr)
  Constant2 : Constant  Value=0.5*mb*g*Lf/(Lf+Lr)+mw*g
  Gain : Gain  Gain=1/mw
  Gain1 : Gain  Gain=kw
  Gain2 : Gain  Gain=kw
  Integrator : Integrator
  Integrator1 : Integrator
  Fzs_rl : Outport
  Fzw_fl : Outport  Port=2
  wires:
  Add5/1 -> Fzs_rl/1
  Constant1/1 -> Add5/2
  Add3/1 -> Add4/2, Add5/1  "F2zs_fl"
  Gain/1 -> Integrator/1
  Add4/1 -> Gain/1
  .1/1 -> Add3/2
  ./1 -> Add3/1
  Add2/1 -> .1/1
  dot_Zs_rl/1 -> Add2/2
  Add1/1 -> ./1
  Zs_rl/1 -> Add1/2
  Add/1 -> Gain1/1
  Integrator1/1 -> Add/1, Add1/1, Add6/2  "Zw_fl"
  Integrator/1 -> Integrator1/1, Add2/1
  Z_road_rl/1 -> Add6/1, Add/2
  Gain1/1 -> Add4/1  "F2zw_fl"
  Add6/1 -> Gain2/1
  Gain2/1 -> Add7/1  "F2zw_fl"
  Constant2/1 -> Add7/2
  Add7/1 -> Fzw_fl/1

== system trucksim_specific_control_with_rule_model/14DOF整车模型/Body/Suspension_Z/rr ==
  dot_Zs_rr : Inport
  Z_road_rr : Inport  Port=2
  Zs_rr : Inport  Port=3
  . : Gain  Gain=ks_f
  .1 : Gain  Gain=Cs_f
  Add : Sum  Inputs=-+
  Add{1..2,4,6} (4 alike) : Sum  Inputs=+-
  Add3 : Sum
  Add5 : Sum
  Add7 : Sum
  Constant1 : Constant  Value=0.5*mb*g*Lf/(Lf+Lr)
  Constant2 : Constant  Value=0.5*mb*g*Lf/(Lf+Lr)+mw*g
  Gain : Gain  Gain=1/mw
  Gain1 : Gain  Gain=kw
  Gain2 : Gain  Gain=kw
  Integrator : Integrator
  Integrator1 : Integrator
  Fzs_rr : Outport
  Fzw_fl : Outport  Port=2
  wires:
  Add5/1 -> Fzs_rr/1
  Constant1/1 -> Add5/2
  Add3/1 -> Add4/2, Add5/1  "F2zs_fl"
  Integrator/1 -> Add2/1, Integrator1/1
  Integrator1/1 -> Add6/2, Add1/1, Add/1  "Zw_fl"
  Add/1 -> Gain1/1
  Zs_rr/1 -> Add1/2
  Add1/1 -> ./1
  dot_Zs_rr/1 -> Add2/2
  Add2/1 -> .1/1
  ./1 -> Add3/1
  .1/1 -> Add3/2
  Add4/1 -> Gain/1
  Gain/1 -> Integrator/1
  Z_road_rr/1 -> Add6/1, Add/2
  Gain1/1 -> Add4/1  "F2zw_fl"
  Add6/1 -> Gain2/1
  Gain2/1 -> Add7/1  "F2zw_fl"
  Constant2/1 -> Add7/2
  Add7/1 -> Fzw_fl/1

== system trucksim_specific_control_with_rule_model/14DOF整车模型/Body/Suspension_Z/zb_to_zs ==
  ddot_phi : Inport
  ddot_theta : Inport  Port=2
  ddot_zb : Inport  Port=3
  Bf/2 : Gain  Gain=0.5*Bf
  Br/2 : Gain  Gain=0.5*Br
  Integrator{,1..3} (4 alike) : Integrator
  Lf : Gain  Gain=Lf
  Lr : Gain  Gain=Lr
  Sum1 : Sum  Inputs=+--
  Sum2 : Sum  Inputs=+++
  Sum3 : Sum  Inputs=+-+
  Sum8 : Sum  Inputs=++-
  dot_Zs_fl : Outport
  dot_Zs_fr : Outport  Port=2
  dot_Zs_rl : Outport  Port=3
  dot_Zs_rr : Outport  Port=4
  wires:
  ddot_phi/1 -> Br/2/1, Bf/2/1
  ddot_theta/1 -> Lr/1, Lf/1
  ddot_zb/1 -> Sum8/1, Sum1/1, Sum3/1, Sum2/1
  Bf/2/1 -> Sum1/2, Sum8/2
  Lf/1 -> Sum1/3, Sum8/3
  Sum8/1 -> Integrator/1
  Sum1/1 -> Integrator1/1
  Br/2/1 -> Sum3/2, Sum2/2
  Lr/1 -> Sum3/3, Sum2/3
  Sum2/1 -> Integrator2/1
  Sum3/1 -> Integrator3/1
  Integrator/1 -> dot_Zs_fl/1
  Integrator1/1 -> dot_Zs_fr/1
  Integrator2/1 -> dot_Zs_rl/1
  Integrator3/1 -> dot_Zs_rr/1

== system trucksim_specific_control_with_rule_model/14DOF整车模型/alpha_lamda/alpha/fl ==
  vx : Inport
  vy : Inport  Port=2
  wz : Inport  Port=3
  delta_fl : Inport  Port=4
  Add2 : Sum
  Add3 : Sum  Inputs=+-
  Add4 : Sum  Inputs=-+
  Divide : Product  Inputs=/*
  Gain3 : Gain  Gain=Lf
  Gain4 : Gain  Gain=0.5*Bf
  Scope : Scope
  Trigonometric Function : Trigonometry  Operator=atan
  alpha_fl : Outport
  wires:
  Gain3/1 -> Add2/2
  Gain4/1 -> Add3/2
  Add2/1 -> Divide/2
  Add3/1 -> Divide/1
  Divide/1 -> Trigonometric Function/1
  Trigonometric Function/1 -> Scope/1, Add4/1
  vx/1 -> Add3/1
  delta_fl/1 -> Add4/2
  vy/1 -> Add2/1
  Add4/1 -> alpha_fl/1
  wz/1 -> Gain4/1, Gain3/1

== system trucksim_specific_control_with_rule_model/14DOF整车模型/alpha_lamda/alpha/fr ==
  vx : Inport
  vy : Inport  Port=2
  wz : Inport  Port=3
  delta_fr : Inport  Port=4
  Add2 : Sum
  Add3 : Sum
  Add4 : Sum  Inputs=-+
  Divide : Product  Inputs=/*
  Gain3 : Gain  Gain=Lf
  Gain4 : Gain  Gain=0.5*Bf
  Trigonometric Function : Trigonometry  Operator=atan
  alpha_fr : Outport
  wires:
  Gain4/1 -> Add3/2
  wz/1 -> Gain3/1, Gain4/1
  Add4/1 -> alpha_fr/1
  vy/1 -> Add2/1
  delta_fr/1 -> Add4/2
  vx/1 -> Add3/1
  Trigonometric Function/1 -> Add4/1
  Divide/1 -> Trigonometric Function/1
  Add3/1 -> Divide/1
  Add2/1 -> Divide/2
  Gain3/1 -> Add2/2

== system trucksim_specific_control_with_rule_model/14DOF整车模型/alpha_lamda/alpha/rl ==
  vx : Inport
  vy : Inport  Port=2
  wz : Inport  Port=3
  delta_rl : Inport  Port=4
  Add2 : Sum  Inputs=+-
  Add3 : Sum  Inputs=+-
  Add4 : Sum  Inputs=-+
  Divide : Product  Inputs=/*
  Gain3 : Gain  Gain=Lr
  Gain4 : Gain  Gain=0.5*Br
  Trigonometric Function : Trigonometry  Operator=atan
  alpha_rl : Outport
  wires:
  Add4/1 -> alpha_rl/1
  Gain4/1 -> Add3/2
  Trigonometric Function/1 -> Add4/1
  wz/1 -> Gain3/1, Gain4/1  "wz"
  vy/1 -> Add2/1  "vy"
  vx/1 -> Add3/1  "vx"
  Divide/1 -> Trigonometric Function/1
  Add3/1 -> Divide/1  "Vx_rl"
  Add2/1 -> Divide/2  "Vy_rl"
  Gain3/1 -> Add2/2
  delta_rl/1 -> Add4/2

== system trucksim_specific_control_with_rule_model/14DOF整车模型/alpha_lamda/alpha/rr ==
  vx : Inport
  vy : Inport  Port=2
  wz : Inport  Port=3
  delta_rr : Inport  Port=4
  Add2 : Sum  Inputs=+-
  Add3 : Sum
  Add4 : Sum  Inputs=-+
  Divide : Product  Inputs=/*
  Gain3 : Gain  Gain=Lr
  Gain4 : Gain  Gain=0.5*Br
  Trigonometric Function : Trigonometry  Operator=atan
  alpha_rr : Outport
  wires:
  Add4/1 -> alpha_rr/1
  Gain4/1 -> Add3/2
  Gain3/1 -> Add2/2
  Add2/1 -> Divide/2  "Vy_rr"
  Add3/1 -> Divide/1  "Vx_rr"
  Divide/1 -> Trigonometric Function/1
  vx/1 -> Add3/1  "vx"
  vy/1 -> Add2/1  "vy"
  wz/1 -> Gain4/1, Gain3/1  "wz"
  Trigonometric Function/1 -> Add4/1
  delta_rr/1 -> Add4/2

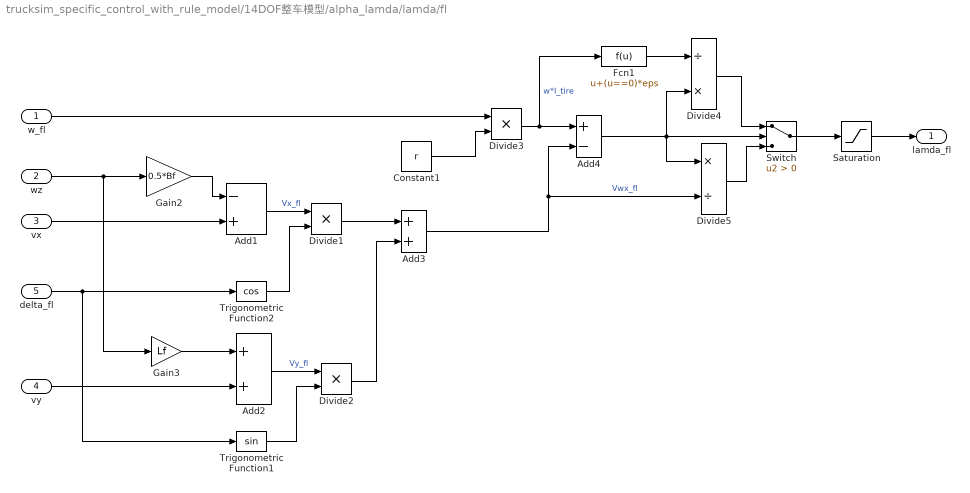
== system trucksim_specific_control_with_rule_model/14DOF整车模型/alpha_lamda/lamda/fl ==
  w_fl : Inport
  wz : Inport  Port=2
  vx : Inport  Port=3
  vy : Inport  Port=4
  delta_fl : Inport  Port=5
  Add1 : Sum  Inputs=-+
  Add2 : Sum
  Add3 : Sum
  Add4 : Sum  Inputs=+-
  Constant1 : Constant  Value=r
  Divide1 : Product  Inputs=**
  Divide2 : Product  Inputs=**
  Divide3 : Product  Inputs=**
  Divide4 : Product  Inputs=/*
  Divide5 : Product  Inputs=*/
  Fcn1 : Fcn  Expr=u+(u==0)*eps
  Gain2 : Gain  Gain=0.5*Bf
  Gain3 : Gain  Gain=Lf
  Saturation : Saturate  UpperLimit=1  LowerLimit=-1
  Switch : Switch  Criteria=u2 > Threshold  SaturateOnIntegerOverflow=off  InputSameDT=off
  Trigonometric Function1 : Trigonometry
  Trigonometric Function2 : Trigonometry  Operator=cos
  lamda_fl : Outport
  wires:
  Saturation/1 -> lamda_fl/1
  Divide3/1 -> Fcn1/1, Add4/1  "w*I_tire"
  Constant1/1 -> Divide3/2
  w_fl/1 -> Divide3/1
  Divide2/1 -> Add3/2
  Divide1/1 -> Add3/1
  Trigonometric Function1/1 -> Divide2/2
  Add2/1 -> Divide2/1  "Vy_fl"
  Gain3/1 -> Add2/1
  vy/1 -> Add2/2
  Trigonometric Function2/1 -> Divide1/2
  delta_fl/1 -> Trigonometric Function1/1, Trigonometric Function2/1
  Add1/1 -> Divide1/1  "Vx_fl"
  wz/1 -> Gain2/1, Gain3/1
  Gain2/1 -> Add1/1
  vx/1 -> Add1/2
  Fcn1/1 -> Divide4/1
  Divide5/1 -> Switch/3
  Divide4/1 -> Switch/1
  Add4/1 -> Divide5/1, Divide4/2, Switch/2
  Add3/1 -> Divide5/2, Add4/2  "Vwx_fl"
  Switch/1 -> Saturation/1
